simulink model "scalar_const_noise_est"  (Simulink 5.0)
settings: Solver=FixedStepDiscrete  SolverMode=SingleTasking  StartTime=0.0  StopTime=100.0  FixedStep=1  RelTol=1e-3
undefined symbols (not defined in the file or in its folder): recursive_avg
libraries: simulink x1
settings Model: Creator=mcarroll  LastModifiedBy=mcarroll  ExtModeAutoUpdateStatusClock=off  BlockReductionOpt=off  BooleanDataType=off  OptimizeBlockIOStorage=off

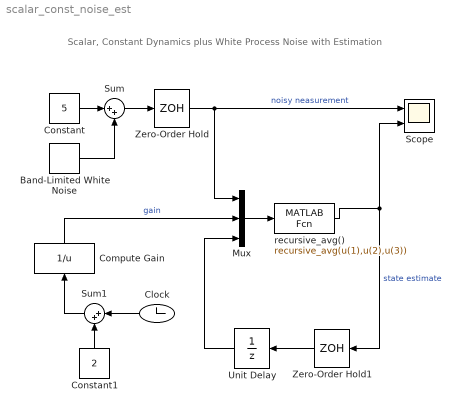
== system scalar_const_noise_est ==
  note: Scalar, Constant Dynamics
      | plus White Process Noise
      | with Estimation
  Band-Limited White Noise : simulink/Sources/Band-Limited White Noise  Cov=[0.1]  Ts=1  seed=[23341+floor(1000*rand(1))]
  Clock : Clock
  Compute Gain : MATLABFcn  Orientation=up  MATLABFcn=1/u  Output1D=off
  Constant : Constant  Value=5
  Constant1 : Constant  Orientation=up  Value=2
  Mux : Mux  Inputs=3
  Scope : Scope  NumInputPorts=2
      settings: YMin=2.5~2.5  YMax=7.5~7.5
  Sum : Sum  Inputs=|++  SaturateOnIntegerOverflow=on  InputSameDT=on
  Sum1 : Sum  Orientation=left  Inputs=|++  SaturateOnIntegerOverflow=on  InputSameDT=on
  Unit Delay : UnitDelay  Orientation=left  SampleTime=-1
  Zero-Order Hold : ZeroOrderHold
  Zero-Order Hold1 : ZeroOrderHold  Orientation=left
  recursive_avg() : MATLABFcn  MATLABFcn=recursive_avg(u(1),u(2),u(3))
  wires:
  Band-Limited White Noise/1 -> Sum/2
  Constant/1 -> Sum/1
  Sum/1 -> Zero-Order Hold/1
  recursive_avg()/1 -> Scope/2, Zero-Order Hold1/1  "state estimate"
  Mux/1 -> recursive_avg()/1
  Clock/1 -> Sum1/1
  Constant1/1 -> Sum1/2
  Sum1/1 -> Compute Gain/1
  Zero-Order Hold/1 -> Scope/1, Mux/1  "noisy neasurement"
  Zero-Order Hold1/1 -> Unit Delay/1
  Compute Gain/1 -> Mux/2  "gain"
  Unit Delay/1 -> Mux/3
